simulink model "SensorlessStartupTest"  (R2026b)
settings: Solver=FixedStepDiscrete  StopTime=startupTestCfg.Duration  FixedStep=startupCfg.Ts
PostLoadFcn:
  | addpath(fullfile(fileparts(get_param(bdroot,'FileName')),'..','build_process'));initialize_startup_test(bdroot);
model workspace (MAT data in the model file):
  startupCfg.Ts = 5e-05
  startupCfg.Theta0 = 0
  startupCfg.AlignCurrent = 2
  startupCfg.StartupCurrent = 3
  startupCfg.FinalOmega = 250
  startupCfg.FlyingCaptureTime = 0.03
  startupCfg.PrealignTime = 0.06
  startupCfg.PrealignRampTime = 0.03
  startupCfg.AlignTime = 0.08
  startupCfg.AlignRampTime = 0.04
  startupCfg.OmegaRampTime = 0.35
  startupCfg.CurrentRampTime = 0.05
  startupCfg.MinCaptureOmega = 150
  startupCfg.MaxIFTime = 0.8
  startupCfg.Samples = [600 1200 600 1600 800 7000 1000 16000]
  startupCfg.Vector = [5e-05; 0; 2; 3; 250; 600; 1200; 600; 1600; 800; 7000; 1000; 16000; 150]
  startupCfg.State0 = [0; 0; 0; 0; 0]
  startupTestCfg.Duration = 1.1
  startupTestCfg.Enable = 1
  startupTestCfg.Reset = 0
  startupTestCfg.Direction = 1
  startupTestCfg.Acquired = 0
  testStim.time = [0 5e-05 0.0001 0.00015 0.0002 0.00025 0.0003 0.00035 0.0004 0.00045 0.0005 0.00055 ... (22001 elements, 22001x1)]
  testStim.signals.values = [1 1 1 1 1 1 1 1 1 1 1 1 ... (88004 elements, 22001x4)]
  testStim.signals.dimensions = 4
libraries: SensorlessStartup x1
settings Model: Creator=24322  LastModifiedBy=24322

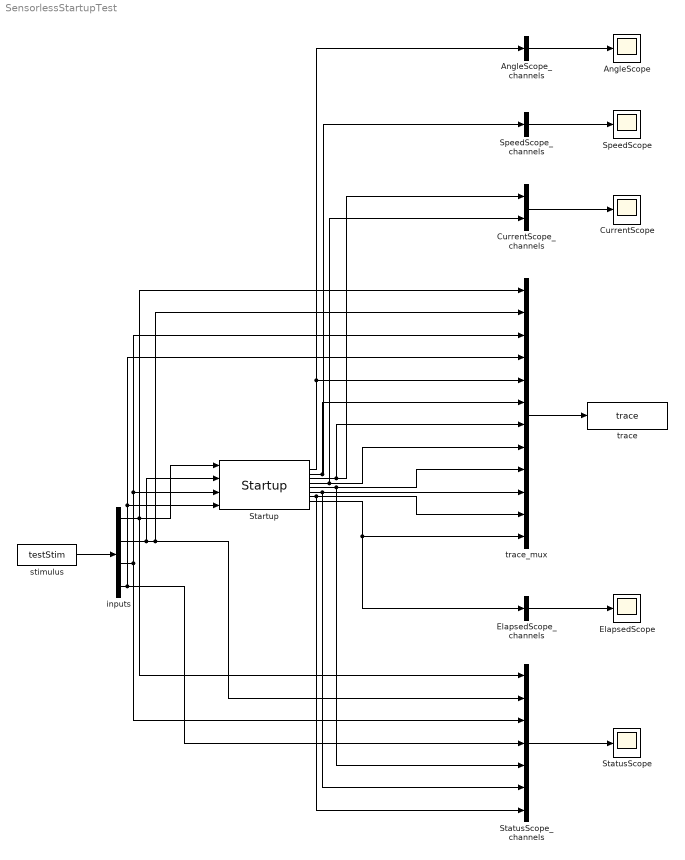
== system SensorlessStartupTest ==
  AngleScope : Scope
  AngleScope_channels : Mux  Inputs=1
  CurrentScope : Scope
  CurrentScope_channels : Mux  Inputs=2
  ElapsedScope : Scope
  ElapsedScope_channels : Mux  Inputs=1
  SpeedScope : Scope
  SpeedScope_channels : Mux  Inputs=1
  Startup : SensorlessStartup/Startup  startupCfg=startupCfg
  StatusScope : Scope
  StatusScope_channels : Mux  Inputs=7
  inputs : Demux
  stimulus : FromWorkspace  VariableName=testStim  SampleTime=startupCfg.Ts  Interpolate=off  OutputAfterFinalValue=Holding final value
  trace : ToWorkspace  VariableName=trace  SaveFormat=Structure With Time  SampleTime=-1
  trace_mux : Mux  Inputs=12
  wires:
  ElapsedScope_channels/1 -> ElapsedScope/1
  StatusScope_channels/1 -> StatusScope/1
  CurrentScope_channels/1 -> CurrentScope/1
  SpeedScope_channels/1 -> SpeedScope/1
  AngleScope_channels/1 -> AngleScope/1
  Startup/8 -> trace_mux/12, ElapsedScope_channels/1
  Startup/7 -> trace_mux/11, StatusScope_channels/7
  Startup/6 -> trace_mux/10, StatusScope_channels/6
  Startup/5 -> trace_mux/9, StatusScope_channels/5
  Startup/4 -> trace_mux/8, CurrentScope_channels/2
  Startup/3 -> trace_mux/7, CurrentScope_channels/1
  Startup/2 -> trace_mux/6, SpeedScope_channels/1
  Startup/1 -> trace_mux/5, AngleScope_channels/1
  inputs/4 -> Startup/4, trace_mux/4, StatusScope_channels/4
  inputs/3 -> trace_mux/3, Startup/3, StatusScope_channels/3
  inputs/2 -> trace_mux/2, StatusScope_channels/2, Startup/2
  inputs/1 -> StatusScope_channels/1, Startup/1, trace_mux/1
  trace_mux/1 -> trace/1
  stimulus/1 -> inputs/1
